simulink model "Robot_V11_DH_Dinamica"  (R2025b)
settings: Solver=ode1  StartTime=0.0  StopTime=5  FixedStep=0.001  RelTol=1e-3
InitFcn:
  | addpath(fileparts(which(bdroot)));
undefined symbols (not defined in the file): X, Y, Z
libraries: sm_lib x28, nesl_utility x27
settings Model: Creator=nnavn  LastModifiedBy=nnavn

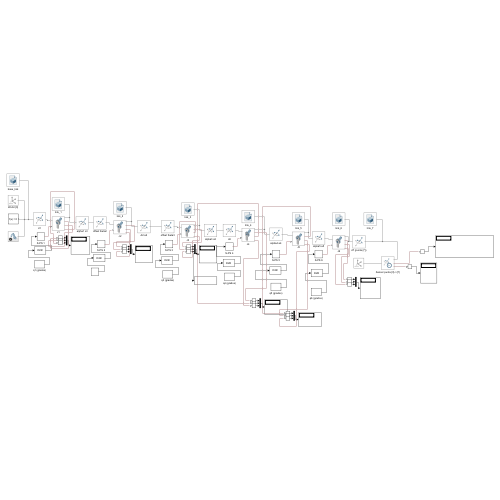
[thumbnail: Simulink's stored preview of the top-level diagram]
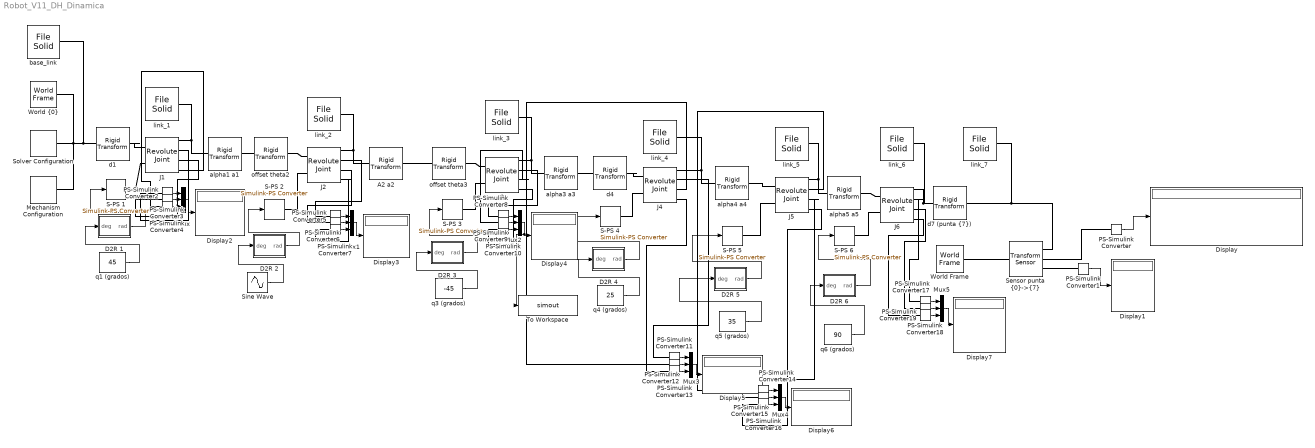
== system Robot_V11_DH_Dinamica ==
  A2 a2 : sm_lib/Frames and Transforms/Rigid Transform  RotationMethod=None  FollAlignAxisA=+X  BaseAlignAxisA=+Y  FollAlignAxisB=+Y  BaseAlignAxisB=+Z  RotationStandardAxis=+Z  RotationAngle=0  RotationAngleUnits=deg  RotationArbitraryAxis=[0 0 1]  RotationSequenceAxes=FollowerAxes  RotationSequence=XYX  RotationSequenceAngles=[0 0 0]  RotationSequenceAnglesUnits=deg  RotationMatrix=[1 0 0;0 1 0;0 0 1]  Quaternion=[1 0 0 0]  TranslationMethod=StandardAxis  TranslationCartesianOffset=[0 0 0]  TranslationCartesianOffsetUnits=m  TranslationStandardAxis=+X  TranslationStandardOffset=0.16  TranslationStandardOffsetUnits=m  TranslationROffset=0  TranslationROffsetUnits=m  TranslationThetaOffset=0  TranslationThetaOffsetUnits=deg  TranslationZOffset=0  TranslationZOffsetUnits=m
  D2R 1 : Subsystem
      mask Display: disp('D2R')
  D2R 2 : Subsystem
      mask Display: disp('D2R')
  D2R 3 : Subsystem
      mask Display: disp('D2R')
  D2R 4 : Subsystem
      mask Display: disp('D2R')
  D2R 5 : Subsystem
      mask Display: disp('D2R')
  D2R 6 : Subsystem
      mask Display: disp('D2R')
  Display{,1..7} (8 alike) : Display
  J{1..6} (6 alike) : sm_lib/Joints/Revolute Joint  JointMode=Normal  CompositeWrenchDir=FollowerOnBase  CompositeWrenchFrame=BaseFrame  SenseConstraintForce=off  SenseConstraintTorque=off  SenseTotalForce=off  SenseTotalTorque=off  PositionTargetSpecify=off  PositionTargetPriority=High  PositionTargetValue=0  PositionTargetValueUnits=deg  VelocityTargetSpecify=off  VelocityTargetPriority=High  VelocityTargetValue=0  VelocityTargetValueUnits=deg/s  EquilibriumPosition=0  EquilibriumPositionUnits=deg  SpringStiffness=0  SpringStiffnessUnits=N*m/deg  DampingCoefficient=0  DampingCoefficientUnits=N*m/(deg/s)  LowerLimitSpecify=off  LowerLimitBound=-90  LowerLimitBoundUnits=deg  LowerLimitStiffness=1e4  LowerLimitStiffnessUnits=N*m/deg  LowerLimitDamping=10  LowerLimitDampingUnits=N*m/(deg/s)  LowerLimitTransitionRegionWidth=0.1  LowerLimitTransitionRegionWidthUnits=deg  UpperLimitSpecify=off  UpperLimitBound=90  UpperLimitBoundUnits=deg  UpperLimitStiffness=1e4  UpperLimitStiffnessUnits=N*m/deg  UpperLimitDamping=10  UpperLimitDampingUnits=N*m/(deg/s)  UpperLimitTransitionRegionWidth=0.1  UpperLimitTransitionRegionWidthUnits=deg  TorqueActuationMode=ComputedTorque  MotionActuationMode=InputMotion  SensePosition=off  SenseVelocity=off  SenseAcceleration=off  SenseTorqueForce=on  SenseLowerLimitTorqueForce=on  SenseUpperLimitTorqueForce=on
  Mechanism Configuration : sm_lib/Utilities/Mechanism Configuration  UniformGravity=Constant  GravityVector=[0 0 -9.81]  GravityVectorUnits=m/s^2  LinearizationDelta=0.001  JointModeTransitionNonlinearIterations=2
  Mux{,1..5} (6 alike) : Mux  Inputs=3
  PS-Simulink Converter{,1..19} (20 alike) : nesl_utility/PS-Simulink Converter  PhysicalDomain=network_engine_domain  SubClassName=ps_output  LeftPortType=input  RightPortType=output  PseudoPeriodic=off  Frequencies=[]  VectorFormat=inherit  Unit=inherit  AffineConversion=off
  S-PS {1..6} (6 alike) : nesl_utility/Simulink-PS Converter  PhysicalDomain=network_engine_domain  SubClassName=ps_input  LeftPortType=input  RightPortType=output  PseudoPeriodic=off  Frequencies=[]  NoiseDistribution=none  NoiseParameters=[]  Unit=rad  AffineConversion=off  FilteringAndDerivatives=filter  SimscapeFilterOrder=2  InputFilterTimeConstant=0.01  UdotUserProvided=0
  "Sensor punta {0}->{7}" : sm_lib/Frames and Transforms/Transform Sensor  MeasurementFrame=World  RotationSequence=XYX  SenseAngle=off  SenseAxis=off  SenseQ=off  SenseR=on  SenseRotationSequence=off  SenseOmegaX=off  SenseOmegaY=off  SenseOmegaZ=off  SenseOmega=off  SenseQDot=off  SenseRDot=off  SenseRotationSequenceDot=off  SenseAlphaX=off  SenseAlphaY=off  SenseAlphaZ=off  SenseAlpha=off  SenseQDDot=off  SenseRDDot=off  SenseX=off  SenseY=off  SenseZ=off  SenseXYZ=on  SenseRad=off  SenseAzim=off  SenseDist=off  SenseInc=off  SenseXDot=off  SenseYDot=off  SenseZDot=off  SenseXYZDot=off  SenseRadDot=off  SenseAzimDot=off  SenseDistDot=off  SenseIncDot=off  SenseXDDot=off  SenseYDDot=off  SenseZDDot=off  SenseXYZDDot=off  SenseRadDDot=off  SenseAzimDDot=off  SenseDistDDot=off  SenseIncDDot=off
  Sine Wave : Sin  Amplitude=90  SampleTime=0
  Solver Configuration : nesl_utility/Solver Configuration  PhysicalDomain=network_engine_domain  SubClassName=solver  LeftPortType=input  RightPortType=generic  Tones=[]  Harmonics=[]  SimulateNoise=off  Profile=off  UseLocalSampling=off  EnableSwitchedLinearOptims=on  FrequencyDomain=off  UseCCode=off  RelTol=0.001  AbsTol=0.001  MinStep=1e-09  ToWorkspace=off  RevertToSquareIcSolve=off  NumHomotopyIterations=100  PhasorMode=off  PhasorModeNumHarmonics=1  ConsistencySolver=NEWTON_XTOL_AFTER_FTOL  IndexReductionMethod=DerivativeReplacement  DoDC=off  ResidualTolerance=1e-09  ConsistencyTolSource=GLOBAL  ConsistencyAbsTol=0.001  ConsistencyRelTol=0.001  ConsistencyTolFactor=0.001  UseLocalSolver=off  LocalSolverChoice=NE_BACKWARD_EULER_ADVANCER  ResolveIndetEquations=on  FunctionEvalNumThread=1  LocalSolverSampleTime=0.001  DoFixedCost=off  MaxNonlinIter=3  MaxModeIter=2  ComputeImpulses=off  ImpulseIterations=2  LinearAlgebra=auto  LinearAlgebraNumThread=0  EquationFormulation=NE_TIME_EF  DelaysMemoryBudget=1024  AutomaticFiltering=on  FilteringTimeConstant=0.001  PartitionStorageMethod=AS_NEEDED  PartitionMemoryBudget=1024  PartitionMethod=ROBUST  MultibodyUseLocalSolver=off  MultibodyLocalSolverChoice=ODE1  MultibodyLocalSolverSampleTime=0.001
  To Workspace : ToWorkspace  VariableName=simout  SampleTime=-1
  World Frame : sm_lib/Frames and Transforms/World Frame
  "World {0}" : sm_lib/Frames and Transforms/World Frame
  alpha1 a1 : sm_lib/Frames and Transforms/Rigid Transform  RotationMethod=StandardAxis  FollAlignAxisA=+X  BaseAlignAxisA=+Y  FollAlignAxisB=+Y  BaseAlignAxisB=+Z  RotationStandardAxis=+X  RotationAngle=pi/2  RotationAngleUnits=rad  RotationArbitraryAxis=[0 0 1]  RotationSequenceAxes=FollowerAxes  RotationSequence=XYX  RotationSequenceAngles=[0 0 0]  RotationSequenceAnglesUnits=deg  RotationMatrix=[1 0 0;0 1 0;0 0 1]  Quaternion=[1 0 0 0]  TranslationMethod=None  TranslationCartesianOffset=[0 0 0]  TranslationCartesianOffsetUnits=m  TranslationStandardAxis=+Z  TranslationStandardOffset=0  TranslationStandardOffsetUnits=m  TranslationROffset=0  TranslationROffsetUnits=m  TranslationThetaOffset=0  TranslationThetaOffsetUnits=deg  TranslationZOffset=0  TranslationZOffsetUnits=m
  alpha3 a3 : sm_lib/Frames and Transforms/Rigid Transform  RotationMethod=StandardAxis  FollAlignAxisA=+X  BaseAlignAxisA=+Y  FollAlignAxisB=+Y  BaseAlignAxisB=+Z  RotationStandardAxis=-X  RotationAngle=pi/2  RotationAngleUnits=rad  RotationArbitraryAxis=[0 0 1]  RotationSequenceAxes=FollowerAxes  RotationSequence=XYX  RotationSequenceAngles=[0 0 0]  RotationSequenceAnglesUnits=deg  RotationMatrix=[1 0 0;0 1 0;0 0 1]  Quaternion=[1 0 0 0]  TranslationMethod=None  TranslationCartesianOffset=[0 0 0]  TranslationCartesianOffsetUnits=m  TranslationStandardAxis=+Z  TranslationStandardOffset=0  TranslationStandardOffsetUnits=m  TranslationROffset=0  TranslationROffsetUnits=m  TranslationThetaOffset=0  TranslationThetaOffsetUnits=deg  TranslationZOffset=0  TranslationZOffsetUnits=m
  alpha4 a4 : sm_lib/Frames and Transforms/Rigid Transform  RotationMethod=StandardAxis  FollAlignAxisA=+X  BaseAlignAxisA=+Y  FollAlignAxisB=+Y  BaseAlignAxisB=+Z  RotationStandardAxis=+X  RotationAngle=pi/2  RotationAngleUnits=rad  RotationArbitraryAxis=[0 0 1]  RotationSequenceAxes=FollowerAxes  RotationSequence=XYX  RotationSequenceAngles=[0 0 0]  RotationSequenceAnglesUnits=deg  RotationMatrix=[1 0 0;0 1 0;0 0 1]  Quaternion=[1 0 0 0]  TranslationMethod=None  TranslationCartesianOffset=[0 0 0]  TranslationCartesianOffsetUnits=m  TranslationStandardAxis=+Z  TranslationStandardOffset=0  TranslationStandardOffsetUnits=m  TranslationROffset=0  TranslationROffsetUnits=m  TranslationThetaOffset=0  TranslationThetaOffsetUnits=deg  TranslationZOffset=0  TranslationZOffsetUnits=m
  alpha5 a5 : sm_lib/Frames and Transforms/Rigid Transform  RotationMethod=StandardAxis  FollAlignAxisA=+X  BaseAlignAxisA=+Y  FollAlignAxisB=+Y  BaseAlignAxisB=+Z  RotationStandardAxis=-X  RotationAngle=pi/2  RotationAngleUnits=rad  RotationArbitraryAxis=[0 0 1]  RotationSequenceAxes=FollowerAxes  RotationSequence=XYX  RotationSequenceAngles=[0 0 0]  RotationSequenceAnglesUnits=deg  RotationMatrix=[1 0 0;0 1 0;0 0 1]  Quaternion=[1 0 0 0]  TranslationMethod=None  TranslationCartesianOffset=[0 0 0]  TranslationCartesianOffsetUnits=m  TranslationStandardAxis=+Z  TranslationStandardOffset=0  TranslationStandardOffsetUnits=m  TranslationROffset=0  TranslationROffsetUnits=m  TranslationThetaOffset=0  TranslationThetaOffsetUnits=deg  TranslationZOffset=0  TranslationZOffsetUnits=m
  base_link : sm_lib/Body Elements/File Solid  ExtGeomFileName=V11_base_link.step  UnitType=FromFile  ExtGeomFileUnits=m  StepReaderType=HEX  ExportConvexHullGeometry=off  InertiaType=Custom  BasedOnType=Mass  Density=1000  DensityUnits=kg/m^3  Mass=3.22978608  MassUnits=kg  CenterOfMass=[-0.00441761 0.00021358 0.04987356]  CenterOfMassUnits=m  MomentsOfInertia=[0.01456918 0.01547730 0.02259753]  MomentsOfInertiaUnits=kg*m^2  ProductsOfInertia=[0 0 0]  ProductsOfInertiaUnits=kg*m^2  GraphicType=FromGeometry  MarkerShape=Sphere  MarkerSize=10  GraphicVisPropType=SimpleVisualProperties  GraphicDiffuseColor=[0.5 0.5 0.5]  GraphicOpacity=1  GraphicSpecularColor=[0.5 0.5 0.5 1.0]  GraphicAmbientColor=[0.15 0.15 0.15 1.0]  GraphicEmissiveColor=[0.0 0.0 0.0 1.0]  GraphicShininess=75  DoExposeReferenceFrame=on  SerializedFrames=<Frames/>
  d1 : sm_lib/Frames and Transforms/Rigid Transform  RotationMethod=None  FollAlignAxisA=+X  BaseAlignAxisA=+Y  FollAlignAxisB=+Y  BaseAlignAxisB=+Z  RotationStandardAxis=+Z  RotationAngle=0  RotationAngleUnits=deg  RotationArbitraryAxis=[0 0 1]  RotationSequenceAxes=FollowerAxes  RotationSequence=XYX  RotationSequenceAngles=[0 0 0]  RotationSequenceAnglesUnits=deg  RotationMatrix=[1 0 0;0 1 0;0 0 1]  Quaternion=[1 0 0 0]  TranslationMethod=StandardAxis  TranslationCartesianOffset=[0 0 0]  TranslationCartesianOffsetUnits=m  TranslationStandardAxis=+Z  TranslationStandardOffset=0.224  TranslationStandardOffsetUnits=m  TranslationROffset=0  TranslationROffsetUnits=m  TranslationThetaOffset=0  TranslationThetaOffsetUnits=deg  TranslationZOffset=0  TranslationZOffsetUnits=m
  d4 : sm_lib/Frames and Transforms/Rigid Transform  RotationMethod=None  FollAlignAxisA=+X  BaseAlignAxisA=+Y  FollAlignAxisB=+Y  BaseAlignAxisB=+Z  RotationStandardAxis=+Z  RotationAngle=0  RotationAngleUnits=deg  RotationArbitraryAxis=[0 0 1]  RotationSequenceAxes=FollowerAxes  RotationSequence=XYX  RotationSequenceAngles=[0 0 0]  RotationSequenceAnglesUnits=deg  RotationMatrix=[1 0 0;0 1 0;0 0 1]  Quaternion=[1 0 0 0]  TranslationMethod=StandardAxis  TranslationCartesianOffset=[0 0 0]  TranslationCartesianOffsetUnits=m  TranslationStandardAxis=+Z  TranslationStandardOffset=0.16  TranslationStandardOffsetUnits=m  TranslationROffset=0  TranslationROffsetUnits=m  TranslationThetaOffset=0  TranslationThetaOffsetUnits=deg  TranslationZOffset=0  TranslationZOffsetUnits=m
  "d7 (punta {7})" : sm_lib/Frames and Transforms/Rigid Transform  RotationMethod=None  FollAlignAxisA=+X  BaseAlignAxisA=+Y  FollAlignAxisB=+Y  BaseAlignAxisB=+Z  RotationStandardAxis=+Z  RotationAngle=0  RotationAngleUnits=deg  RotationArbitraryAxis=[0 0 1]  RotationSequenceAxes=FollowerAxes  RotationSequence=XYX  RotationSequenceAngles=[0 0 0]  RotationSequenceAnglesUnits=deg  RotationMatrix=[1 0 0;0 1 0;0 0 1]  Quaternion=[1 0 0 0]  TranslationMethod=StandardAxis  TranslationCartesianOffset=[0 0 0]  TranslationCartesianOffsetUnits=m  TranslationStandardAxis=+Z  TranslationStandardOffset=0.085  TranslationStandardOffsetUnits=m  TranslationROffset=0  TranslationROffsetUnits=m  TranslationThetaOffset=0  TranslationThetaOffsetUnits=deg  TranslationZOffset=0  TranslationZOffsetUnits=m
  link_1 : sm_lib/Body Elements/File Solid  ExtGeomFileName=V11_link_1.step  UnitType=FromFile  ExtGeomFileUnits=m  StepReaderType=HEX  ExportConvexHullGeometry=off  InertiaType=Custom  BasedOnType=Mass  Density=1000  DensityUnits=kg/m^3  Mass=1.42277105  MassUnits=kg  CenterOfMass=|  CenterOfMassUnits=m  MomentsOfInertia=[0.00355071 0.00349208 0.00176143]  MomentsOfInertiaUnits=kg*m^2  ProductsOfInertia=[0 0 0]  ProductsOfInertiaUnits=kg*m^2  GraphicType=FromGeometry  MarkerShape=Sphere  MarkerSize=10  GraphicVisPropType=SimpleVisualProperties  GraphicDiffuseColor=[0.5 0.5 0.5]  GraphicOpacity=1  GraphicSpecularColor=[0.5 0.5 0.5 1.0]  GraphicAmbientColor=[0.15 0.15 0.15 1.0]  GraphicEmissiveColor=[0.0 0.0 0.0 1.0]  GraphicShininess=75  DoExposeReferenceFrame=on  SerializedFrames=<Frames/>
      | [0.00002116 -0.00249327 -0.02470983
      | ]
  link_2 : sm_lib/Body Elements/File Solid  ExtGeomFileName=V11_link_2.step  UnitType=FromFile  ExtGeomFileUnits=m  StepReaderType=HEX  ExportConvexHullGeometry=off  InertiaType=Custom  BasedOnType=Mass  Density=1000  DensityUnits=kg/m^3  Mass=1.25185199  MassUnits=kg  CenterOfMass=[0.11123543 0.00005934 -0.00470450]  CenterOfMassUnits=m  MomentsOfInertia=[0.00211573 0.00696012 0.00548348]  MomentsOfInertiaUnits=kg*m^2  ProductsOfInertia=[0 0 0]  ProductsOfInertiaUnits=kg*m^2  GraphicType=FromGeometry  MarkerShape=Sphere  MarkerSize=10  GraphicVisPropType=SimpleVisualProperties  GraphicDiffuseColor=[0.5 0.5 0.5]  GraphicOpacity=1  GraphicSpecularColor=[0.5 0.5 0.5 1.0]  GraphicAmbientColor=[0.15 0.15 0.15 1.0]  GraphicEmissiveColor=[0.0 0.0 0.0 1.0]  GraphicShininess=75  DoExposeReferenceFrame=on  SerializedFrames=<Frames/>
  link_3 : sm_lib/Body Elements/File Solid  ExtGeomFileName=V11_link_3.step  UnitType=FromFile  ExtGeomFileUnits=m  StepReaderType=HEX  ExportConvexHullGeometry=off  InertiaType=Custom  BasedOnType=Mass  Density=1000  DensityUnits=kg/m^3  Mass=0.58966599  MassUnits=kg  CenterOfMass=|  CenterOfMassUnits=m  MomentsOfInertia=|  MomentsOfInertiaUnits=kg*m^2  ProductsOfInertia=[0 0 0]  ProductsOfInertiaUnits=kg*m^2  GraphicType=FromGeometry  MarkerShape=Sphere  MarkerSize=10  GraphicVisPropType=SimpleVisualProperties  GraphicDiffuseColor=[0.5 0.5 0.5]  GraphicOpacity=1  GraphicSpecularColor=[0.5 0.5 0.5 1.0]  GraphicAmbientColor=[0.15 0.15 0.15 1.0]  GraphicEmissiveColor=[0.0 0.0 0.0 1.0]  GraphicShininess=75  DoExposeReferenceFrame=on  SerializedFrames=<Frames/>
      CenterOfMass=|
      | [ -0.00009416
      |  0.04213010
      |  -0.00460755]
      MomentsOfInertia=|
      | [0.00170461 0.00133106 0.00063002
      | ]
  link_4 : sm_lib/Body Elements/File Solid  ExtGeomFileName=V11_link_4.step  UnitType=FromFile  ExtGeomFileUnits=m  StepReaderType=HEX  ExportConvexHullGeometry=off  InertiaType=Custom  BasedOnType=Mass  Density=1000  DensityUnits=kg/m^3  Mass=0.47958111  MassUnits=kg  CenterOfMass=|  CenterOfMassUnits=m  MomentsOfInertia="[0.00072785  0.00066618 0.00040986]"  MomentsOfInertiaUnits=kg*m^2  ProductsOfInertia=[0 0 0]  ProductsOfInertiaUnits=kg*m^2  GraphicType=FromGeometry  MarkerShape=Sphere  MarkerSize=10  GraphicVisPropType=SimpleVisualProperties  GraphicDiffuseColor=[0.5 0.5 0.5]  GraphicOpacity=1  GraphicSpecularColor=[0.5 0.5 0.5 1.0]  GraphicAmbientColor=[0.15 0.15 0.15 1.0]  GraphicEmissiveColor=[0.0 0.0 0.0 1.0]  GraphicShininess=75  DoExposeReferenceFrame=on  SerializedFrames=<Frames/>
      | [-0.00008520
      | -0.00067765
      | -0.02985032]
  link_5 : sm_lib/Body Elements/File Solid  ExtGeomFileName=V11_link_5.step  UnitType=FromFile  ExtGeomFileUnits=m  StepReaderType=HEX  ExportConvexHullGeometry=off  InertiaType=Custom  BasedOnType=Mass  Density=1000  DensityUnits=kg/m^3  Mass=0.44332189  MassUnits=kg  CenterOfMass=|  CenterOfMassUnits=m  MomentsOfInertia=[0.00057612 0.00037214 0.00034469]  MomentsOfInertiaUnits=kg*m^2  ProductsOfInertia=[0 0 0]  ProductsOfInertiaUnits=kg*m^2  GraphicType=FromGeometry  MarkerShape=Sphere  MarkerSize=10  GraphicVisPropType=SimpleVisualProperties  GraphicDiffuseColor=[0.5 0.5 0.5]  GraphicOpacity=1  GraphicSpecularColor=[0.5 0.5 0.5 1.0]  GraphicAmbientColor=[0.15 0.15 0.15 1.0]  GraphicEmissiveColor=[0.0 0.0 0.0 1.0]  GraphicShininess=75  DoExposeReferenceFrame=on  SerializedFrames=<Frames/>
      | [ -0.00010871
      | 0.03642818
      | -0.00232872]
  link_6 : sm_lib/Body Elements/File Solid  ExtGeomFileName=V11_link_6.step  UnitType=FromFile  ExtGeomFileUnits=m  StepReaderType=HEX  ExportConvexHullGeometry=off  InertiaType=Custom  BasedOnType=Mass  Density=1000  DensityUnits=kg/m^3  Mass=0.05458529  MassUnits=kg  CenterOfMass=|  CenterOfMassUnits=m  MomentsOfInertia=[0.00001352 0.00001352 0.00002663]  MomentsOfInertiaUnits=kg*m^2  ProductsOfInertia=[0 0 0]  ProductsOfInertiaUnits=kg*m^2  GraphicType=FromGeometry  MarkerShape=Sphere  MarkerSize=10  GraphicVisPropType=SimpleVisualProperties  GraphicDiffuseColor=[0.5 0.5 0.5]  GraphicOpacity=1  GraphicSpecularColor=[0.5 0.5 0.5 1.0]  GraphicAmbientColor=[0.15 0.15 0.15 1.0]  GraphicEmissiveColor=[0.0 0.0 0.0 1.0]  GraphicShininess=75  DoExposeReferenceFrame=on  SerializedFrames=<Frames/>
      | [0.00000000
      | 0.00000000
      | 0.08009328]
  link_7 : sm_lib/Body Elements/File Solid  ExtGeomFileName=V11_link_6.step  UnitType=FromFile  ExtGeomFileUnits=m  StepReaderType=HEX  ExportConvexHullGeometry=off  InertiaType=Custom  BasedOnType=Mass  Density=1000  DensityUnits=kg/m^3  Mass=0.5  MassUnits=kg  CenterOfMass=|  CenterOfMassUnits=m  MomentsOfInertia=[0.00001352 0.00001352 0.00002663]  MomentsOfInertiaUnits=kg*m^2  ProductsOfInertia=[0 0 0]  ProductsOfInertiaUnits=kg*m^2  GraphicType=FromGeometry  MarkerShape=Sphere  MarkerSize=10  GraphicVisPropType=SimpleVisualProperties  GraphicDiffuseColor=[0.5 0.5 0.5]  GraphicOpacity=1  GraphicSpecularColor=[0.5 0.5 0.5 1.0]  GraphicAmbientColor=[0.15 0.15 0.15 1.0]  GraphicEmissiveColor=[0.0 0.0 0.0 1.0]  GraphicShininess=75  DoExposeReferenceFrame=on  SerializedFrames=<Frames/>
      | [0.00000000
      | 0.00000000
      | 0.08009328]
  offset theta2 : sm_lib/Frames and Transforms/Rigid Transform  RotationMethod=StandardAxis  FollAlignAxisA=+X  BaseAlignAxisA=+Y  FollAlignAxisB=+Y  BaseAlignAxisB=+Z  RotationStandardAxis=+Z  RotationAngle=pi/2  RotationAngleUnits=rad  RotationArbitraryAxis=[0 0 1]  RotationSequenceAxes=FollowerAxes  RotationSequence=XYX  RotationSequenceAngles=[0 0 0]  RotationSequenceAnglesUnits=deg  RotationMatrix=[1 0 0;0 1 0;0 0 1]  Quaternion=[1 0 0 0]  TranslationMethod=None  TranslationCartesianOffset=[0 0 0]  TranslationCartesianOffsetUnits=m  TranslationStandardAxis=+Z  TranslationStandardOffset=0  TranslationStandardOffsetUnits=m  TranslationROffset=0  TranslationROffsetUnits=m  TranslationThetaOffset=0  TranslationThetaOffsetUnits=deg  TranslationZOffset=0  TranslationZOffsetUnits=m
  offset theta3 : sm_lib/Frames and Transforms/Rigid Transform  RotationMethod=StandardAxis  FollAlignAxisA=+X  BaseAlignAxisA=+Y  FollAlignAxisB=+Y  BaseAlignAxisB=+Z  RotationStandardAxis=-Z  RotationAngle=pi/2  RotationAngleUnits=rad  RotationArbitraryAxis=[0 0 1]  RotationSequenceAxes=FollowerAxes  RotationSequence=XYX  RotationSequenceAngles=[0 0 0]  RotationSequenceAnglesUnits=deg  RotationMatrix=[1 0 0;0 1 0;0 0 1]  Quaternion=[1 0 0 0]  TranslationMethod=None  TranslationCartesianOffset=[0 0 0]  TranslationCartesianOffsetUnits=m  TranslationStandardAxis=+Z  TranslationStandardOffset=0  TranslationStandardOffsetUnits=m  TranslationROffset=0  TranslationROffsetUnits=m  TranslationThetaOffset=0  TranslationThetaOffsetUnits=deg  TranslationZOffset=0  TranslationZOffsetUnits=m
  q1 (grados) : Constant  Value=45
  q3 (grados) : Constant  Value=-45
  q4 (grados) : Constant  Value=25
  q5 (grados) : Constant  Value=35
  q6 (grados) : Constant  Value=90
  wires:
  q1 (grados)/1 -> D2R 1/1(deg)
  D2R 1/1(rad) -> S-PS 1/1
  D2R 2/1(rad) -> S-PS 2/1
  q3 (grados)/1 -> D2R 3/1(deg)
  D2R 3/1(rad) -> S-PS 3/1
  q4 (grados)/1 -> D2R 4/1(deg)
  D2R 4/1(rad) -> S-PS 4/1
  q5 (grados)/1 -> D2R 5/1(deg)
  D2R 5/1(rad) -> S-PS 5/1
  q6 (grados)/1 -> D2R 6/1(deg)
  D2R 6/1(rad) -> S-PS 6/1
  PS-Simulink Converter1/1 -> Display1/1
  PS-Simulink Converter/1 -> Display/1
  PS-Simulink Converter4/1 -> Mux/3
  PS-Simulink Converter3/1 -> Mux/2
  PS-Simulink Converter2/1 -> Mux/1
  Mux/1 -> Display2/1
  PS-Simulink Converter7/1 -> Mux1/3
  Mux1/1 -> Display3/1
  PS-Simulink Converter6/1 -> Mux1/2
  PS-Simulink Converter5/1 -> Mux1/1
  Mux2/1 -> To Workspace/1, Display4/1
  PS-Simulink Converter9/1 -> Mux2/2
  PS-Simulink Converter10/1 -> Mux2/3
  PS-Simulink Converter8/1 -> Mux2/1
  Mux3/1 -> Display5/1
  PS-Simulink Converter12/1 -> Mux3/2
  PS-Simulink Converter13/1 -> Mux3/3
  PS-Simulink Converter11/1 -> Mux3/1
  Mux4/1 -> Display6/1
  PS-Simulink Converter15/1 -> Mux4/2
  PS-Simulink Converter16/1 -> Mux4/3
  PS-Simulink Converter14/1 -> Mux4/1
  Mux5/1 -> Display7/1
  PS-Simulink Converter18/1 -> Mux5/2
  PS-Simulink Converter19/1 -> Mux5/3
  PS-Simulink Converter17/1 -> Mux5/1
  Sine Wave/1 -> D2R 2/1(deg)
  connections:
  Solver Configuration/RConn1 -- "World {0}"/RConn1 -- Mechanism Configuration/RConn1 -- base_link/RConn1 -- d1/LConn1
  d1/RConn1 -- J1/LConn1
  J1/RConn1 -- alpha1 a1/LConn1 -- link_1/RConn1
  S-PS 1/RConn1 -- J1/LConn2
  alpha1 a1/RConn1 -- offset theta2/LConn1
  offset theta2/RConn1 -- J2/LConn1
  J2/RConn1 -- A2 a2/LConn1 -- link_2/RConn1
  S-PS 2/RConn1 -- J2/LConn2
  A2 a2/RConn1 -- offset theta3/LConn1
  offset theta3/RConn1 -- J3/LConn1
  J3/RConn1 -- alpha3 a3/LConn1 -- link_3/RConn1
  S-PS 3/RConn1 -- J3/LConn2
  alpha3 a3/RConn1 -- d4/LConn1
  d4/RConn1 -- J4/LConn1
  J4/RConn1 -- alpha4 a4/LConn1 -- link_4/RConn1
  S-PS 4/RConn1 -- J4/LConn2
  alpha4 a4/RConn1 -- J5/LConn1
  S-PS 5/RConn1 -- J5/LConn2
  alpha5 a5/RConn1 -- J6/LConn1
  J6/RConn1 -- link_6/RConn1 -- "d7 (punta {7})"/LConn1
  S-PS 6/RConn1 -- J6/LConn2
  "d7 (punta {7})"/RConn1 -- link_7/RConn1 -- "Sensor punta {0}->{7}"/RConn1
  link_5/RConn1 -- alpha5 a5/LConn1 -- J5/RConn1
  PS-Simulink Converter/LConn1 -- "Sensor punta {0}->{7}"/RConn2
  "Sensor punta {0}->{7}"/RConn3 -- PS-Simulink Converter1/LConn1
  World Frame/RConn1 -- "Sensor punta {0}->{7}"/LConn1
  J1/RConn2 -- PS-Simulink Converter2/LConn1
  J1/RConn3 -- PS-Simulink Converter3/LConn1
  J1/RConn4 -- PS-Simulink Converter4/LConn1
  J6/RConn2 -- PS-Simulink Converter17/LConn1
  J6/RConn3 -- PS-Simulink Converter18/LConn1
  J6/RConn4 -- PS-Simulink Converter19/LConn1
  J5/RConn2 -- PS-Simulink Converter14/LConn1
  J5/RConn3 -- PS-Simulink Converter15/LConn1
  J5/RConn4 -- PS-Simulink Converter16/LConn1
  J4/RConn2 -- PS-Simulink Converter11/LConn1
  J4/RConn3 -- PS-Simulink Converter12/LConn1
  J4/RConn4 -- PS-Simulink Converter13/LConn1
  J3/RConn2 -- PS-Simulink Converter8/LConn1
  J3/RConn3 -- PS-Simulink Converter9/LConn1
  J3/RConn4 -- PS-Simulink Converter10/LConn1
  J2/RConn2 -- PS-Simulink Converter5/LConn1
  J2/RConn3 -- PS-Simulink Converter6/LConn1
  J2/RConn4 -- PS-Simulink Converter7/LConn1

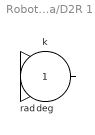
== system Robot_V11_DH_Dinamica/D2R 1 ==
  deg : Inport
  k : Gain  Gain=pi/180
  rad : Outport
  wires:
  deg/1 -> k/1
  k/1 -> rad/1

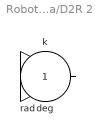
== system Robot_V11_DH_Dinamica/D2R 2 ==
  deg : Inport
  k : Gain  Gain=pi/180
  rad : Outport
  wires:
  deg/1 -> k/1
  k/1 -> rad/1

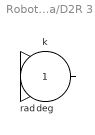
== system Robot_V11_DH_Dinamica/D2R 3 ==
  deg : Inport
  k : Gain  Gain=pi/180
  rad : Outport
  wires:
  deg/1 -> k/1
  k/1 -> rad/1

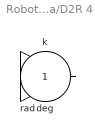
== system Robot_V11_DH_Dinamica/D2R 4 ==
  deg : Inport
  k : Gain  Gain=pi/180
  rad : Outport
  wires:
  deg/1 -> k/1
  k/1 -> rad/1

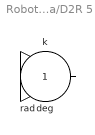
== system Robot_V11_DH_Dinamica/D2R 5 ==
  deg : Inport
  k : Gain  Gain=pi/180
  rad : Outport
  wires:
  deg/1 -> k/1
  k/1 -> rad/1

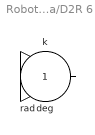
== system Robot_V11_DH_Dinamica/D2R 6 ==
  deg : Inport
  k : Gain  Gain=pi/180
  rad : Outport
  wires:
  deg/1 -> k/1
  k/1 -> rad/1
